simulink model "power_network_model"  (R2024b)
settings: Solver=FixedStepDiscrete  StartTime=0.0  StopTime=0.12  FixedStep=5e-5  RelTol=1e-3
libraries: spsThreePhasePISectionLineLib x2, spsThreePhaseSourceLib x2, spsThreePhaseFaultLib x1, spsThreePhaseVIMeasurementLib x1, spspowerguiLib x1
settings Model: Creator=KRISH PRASAD  LastModifiedBy=KRISH PRASAD

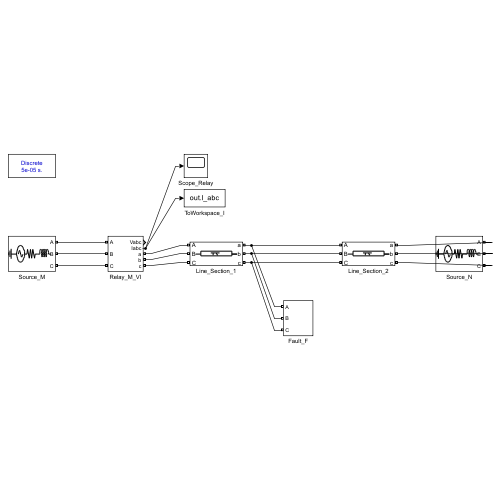
[thumbnail: Simulink's stored preview of the top-level diagram]
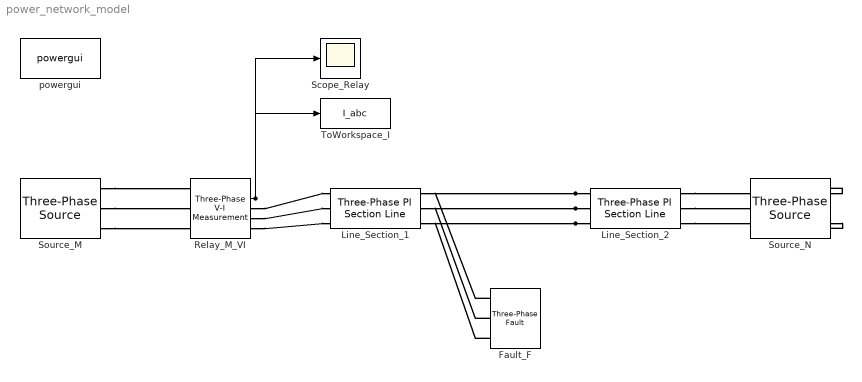
== system power_network_model ==
  Fault_F : spsThreePhaseFaultLib/Three-Phase Fault  InitialStates=0  FaultA=on  FaultB=off  FaultC=off  GroundFault=on  SwitchTimes=[0.04 0.10]  External=off  SwitchStatus=NaN  FaultResistance=0.5  GroundResistance=0.01  SnubberResistance=1e6  SnubberCapacitance=inf  Measurements=None
  Line_Section_1 : spsThreePhasePISectionLineLib/Three-Phase PI Section Line  LConnTagsString=a|b|c  RConnTagsString=A|B|C  Length=30  Frequency=50  Resistances=[0.02, 0.10645]  Inductances=[0.91285e-3, 2.6642e-3]  Capacitances=[14.0e-9, 7.75e-9]
  Line_Section_2 : spsThreePhasePISectionLineLib/Three-Phase PI Section Line  LConnTagsString=a|b|c  RConnTagsString=A|B|C  Length=90  Frequency=50  Resistances=[0.02, 0.10645]  Inductances=[0.91285e-3, 2.6642e-3]  Capacitances=[14.0e-9, 7.75e-9]
  Relay_M_VI : spsThreePhaseVIMeasurementLib/Three-Phase V-I Measurement  VoltageMeasurement=phase-to-ground  SetLabelV=off  LabelV=Vabc  Vpu=off  VpuLL=off  CurrentMeasurement=yes  SetLabelI=off  LabelI=Iabc  Ipu=off  Pbase=100e6  Vbase=500e3  OutputType=Complex  PhasorSimulation=off  PSBequivalent=0
  Scope_Relay : Scope
  Source_M : spsThreePhaseSourceLib/Three-Phase Source  InternalConnection=Yg  VoltagePhases=off  Voltage=230e3  PhaseAngle=0  Voltage_phases=[25e3 25e3 25e3]/sqrt(3)  PhaseAngles_phases=[0 -120 +120]  Frequency=50  NonIdealSource=on  SpecifyImpedance=on  Resistance=0.5  Inductance=0.0159  ShortCircuitLevel=100e6  BaseVoltage=25e3  XRratio=7  BusType=swing  Pref=10e3  Qref=0  Prefabc=[10e3, 10e3, 10e3]  Qrefabc=[0, 0, 0]  Qmin=-inf  Qmax=inf
  Source_N : spsThreePhaseSourceLib/Three-Phase Source  InternalConnection=Yg  VoltagePhases=off  Voltage=230e3  PhaseAngle=-10  Voltage_phases=[25e3 25e3 25e3]/sqrt(3)  PhaseAngles_phases=[0 -120 +120]  Frequency=50  NonIdealSource=on  SpecifyImpedance=on  Resistance=0.5  Inductance=0.0159  ShortCircuitLevel=100e6  BaseVoltage=25e3  XRratio=7  BusType=swing  Pref=10e3  Qref=0  Prefabc=[10e3, 10e3, 10e3]  Qrefabc=[0, 0, 0]  Qmin=-inf  Qmax=inf
  ToWorkspace_I : ToWorkspace  VariableName=I_abc  SampleTime=1e-3
  powergui : spspowerguiLib/powergui  Priority=1  SimulationMode=Discrete  SampleTime=5e-5  frequency=60  Iterations=50  frequencyindice=60  Pbase=100e6  ErrMax=1e-4  UnitsV=kV  UnitsW=MW  buscounter=0  FunctionMessages=off  echomessages=off  EnableUseOfTLC=off  CurrentSourceSwitches=off  DisableSnubberDevices=off  DisableRonSwitches=off  DisableVfSwitches=off  DisplayEquations=off  AutomaticDiscreteSolvers=off  SolverType=Tustin/Backward Euler (TBE)  Interpol=off  ExternalGateDelay=off  methode=off  Ts=100  x0status=blocks  SPID=on  SwTol=0  HookPort=off  NonlinearTolerance=1e-4  nMaxIteration=100  ContinueOnMaxIteration=off  RestoreLinks=warning  ResistiveCurrentMeasurement=off  Frange=[0:2:500]  Ylog=off  Xlog=on  ShowGrid=off  save=off  variable=ZData  structure=0  ZoomFFT=off  StartTime=0.0  cycles=1  DisplayStyle=1  fundamental=60  FreqAxis=off  MaxFrequency=1000  frequencyindicesteady=1  RmsSteady=1  display=off
  wires:
  Relay_M_VI/2 -> ToWorkspace_I/1, Scope_Relay/1
  connections:
  Source_M/RConn1 -- Relay_M_VI/LConn1
  Source_M/RConn2 -- Relay_M_VI/LConn2
  Source_M/RConn3 -- Relay_M_VI/LConn3
  Relay_M_VI/RConn1 -- Line_Section_1/LConn1
  Relay_M_VI/RConn2 -- Line_Section_1/LConn2
  Relay_M_VI/RConn3 -- Line_Section_1/LConn3
  Line_Section_2/LConn1 -- Line_Section_1/RConn1 -- Fault_F/LConn1
  Line_Section_2/LConn2 -- Line_Section_1/RConn2 -- Fault_F/LConn2
  Line_Section_2/LConn3 -- Line_Section_1/RConn3 -- Fault_F/LConn3
  Line_Section_2/RConn1 -- Source_N/RConn1
  Line_Section_2/RConn2 -- Source_N/RConn2
  Line_Section_2/RConn3 -- Source_N/RConn3
